simulink model "arducopter"  (R2021a)
settings: Solver=FixedStepAuto  StartTime=0.0  StopTime=simIn.param.timeEnd  FixedStep=simIn.param.dt  RelTol=1e-3
undefined symbols (not defined in the file or in its folder): DiscIntNeverNeededParam, sim, simIn
libraries: simulink x35, slident x4, vrlib x1
(part 7 of 9)

== matlab function arducopter/Attitude Controller/input_euler_angle_roll_pitch_euler_rate_yaw()/Feedforward enabled/input shaping/input shaping roll angle/Square Root Controller1/Square Root Controller ==
  data: err input; correction_rate output; p input; second_ord_lim input; dt input
function correction_rate = sqrt_controller(err, p, second_ord_lim, dt)
% The square root controller
% Code is taken from sqrt_controller(...) in AC_PosControl.cpp.

if (second_ord_lim < 0 || second_ord_lim == 0)
   correction_rate = err * p;
elseif (p == 0)
    % P term is zero, but second order limit is positive
    if (err > 0)
        correction_rate = sqrt(single(2.0) * second_ord_lim * err);
    elseif (err < 0)
        correction_rate = sqrt(single(2.0) * second_ord_lim * -err);
    else
        correction_rate = single(0.0);
    end
else
    % P term and second order limit are positive, hence have been defined
    linear_dist = second_ord_lim / (p * p);
    % Check if error exceeds linear range of controller gain
    if (err > linear_dist)
        correction_rate = sqrt(single(2.0) * second_ord_lim * ( err - (linear_dist / single(2.0)) ));
    elseif (err < -linear_dist)
        correction_rate = -sqrt(single(2.0) * second_ord_lim * ( -err - (linear_dist / single(2.0)) ));
    else
        % Return linearly amplified correction if error is in linear range
        correction_rate = err * p;
    end
end

% Prevent oscillations by over-shooting the error correction in the last
% time step
if (dt ~= 0)
    correction_rate = max( min(correction_rate, abs(err) / dt), -abs(err) / dt);
end

== matlab function arducopter/Attitude Controller/input_euler_angle_roll_pitch_euler_rate_yaw()/Feedforward enabled/input shaping/input shaping yaw rate/Square Root Controller/Square Root Controller ==
  data: err input; correction_rate output; p input; second_ord_lim input; dt input
function correction_rate = sqrt_controller(err, p, second_ord_lim, dt)
% The square root controller
% Code is taken from sqrt_controller(...) in AC_PosControl.cpp.

if (second_ord_lim < 0 || second_ord_lim == 0)
   correction_rate = err * p;
elseif (p == 0)
    % P term is zero, but second order limit is positive
    if (err > 0)
        correction_rate = sqrt(single(2.0) * second_ord_lim * err);
    elseif (err < 0)
        correction_rate = sqrt(single(2.0) * second_ord_lim * -err);
    else
        correction_rate = single(0.0);
    end
else
    % P term and second order limit are positive, hence have been defined
    linear_dist = second_ord_lim / (p * p);
    % Check if error exceeds linear range of controller gain
    if (err > linear_dist)
        correction_rate = sqrt(single(2.0) * second_ord_lim * ( err - (linear_dist / single(2.0)) ));
    elseif (err < -linear_dist)
        correction_rate = -sqrt(single(2.0) * second_ord_lim * ( -err - (linear_dist / single(2.0)) ));
    else
        % Return linearly amplified correction if error is in linear range
        correction_rate = err * p;
    end
end

% Prevent oscillations by over-shooting the error correction in the last
% time step
if (dt ~= 0)
    correction_rate = max( min(correction_rate, abs(err) / dt), -abs(err) / dt);
end

== matlab function arducopter/Throttle/Throttle Calculations/Throttle-Attitude-Mixing/get_throttle_hover/MATLAB Function ==
  data: thrHover input; thrHoverLim output; thrHoverMin input; thrHoverMax input
function thrHoverLim = constrain(thrHover, thrHoverMin, thrHoverMax)

thrHoverLim = min( max( thrHover, thrHoverMin), thrHoverMax);

== matlab function arducopter/Attitude Controller/Determine angleLimit/MATLAB Function2 ==
  data: altholdLeanAngleMax input; altholdLeanAngleMaxCDeg output; angleLimitMin input
function altholdLeanAngleMaxCDeg = get_althold_lean_angle_max_cd(altholdLeanAngleMax, angleLimitMin)
% Based on AC_AttitudeControl::get_althold_lean_angle_max_cd().
% Function calculates a tilt angle limit for pilot input that prioritises
% altitude hold over lean angle.
altholdLeanAngleMaxCDeg = max(180/pi * altholdLeanAngleMax, angleLimitMin) * 100;

== matlab function arducopter/Throttle/Throttle Calculations/MATLAB Function ==
  data: thrThstMax input; throttle_in input; angleLimitTc input; dt input; angleLimitThrMax input; altholdLeanAngleMax_ data_store_memory; altholdLeanAngleMax output
function altholdLeanAngleMax = update_althold_lean_angle_max(thrThstMax, throttle_in, angleLimitTc, dt, angleLimitThrMax)
% Based on AC_AttitudeControl_Multi::update_althold_lean_angle_max. 
% Function updates Althold angle maximum.

global altholdLeanAngleMax_

if thrThstMax == 0
    altholdLeanAngleMax_ = single(0);
    altholdLeanAngleMax = single(0);
    return;
end

altholdLeanAngleMax = acos(min(max(throttle_in / (angleLimitThrMax * thrThstMax), single(0)), single(1)));
altholdLeanAngleMax_ = altholdLeanAngleMax_ + (dt / (dt + angleLimitTc)) * (altholdLeanAngleMax - altholdLeanAngleMax_);
altholdLeanAngleMax = altholdLeanAngleMax_;

== matlab function arducopter/Throttle/Throttle Calculations/Throttle Limiting based on battery state/Update Lift Max from Battery Voltage ==
  data: battVoltFiltLast input; battVoltFilt output single; battVoltRestEst input; liftMax output single; battVoltMax input; battVoltMin input single; thstCurveExpo input; battVoltMinAct output single; battVoltRestEstAct output single; loop_rate input
function [battVoltFilt, liftMax, battVoltMinAct, battVoltRestEstAct] = update_lift_max_from_batt_voltage(battVoltFiltLast, battVoltRestEst, battVoltMax, battVoltMin, thstCurveExpo, loop_rate)
% Code taken from AP_MotorsMulticopter::update_lift_max_from_batt_voltage()
% in AP_MotorsMulticopter.cpp

% Check if batt_volt_min is too small
if (battVoltMax <= 0 || (battVoltMin >= battVoltMax) ...
        || battVoltRestEst < 0.25 * battVoltMin)
    battVoltFilt = single(1.0);
    liftMax = single(1.0);
    battVoltMinAct = battVoltMin;
    battVoltRestEstAct = battVoltRestEst;
    return;
end

% Set lower battery voltage limit for thrust scaling to a new value
battVoltMinAct = max(battVoltMin, battVoltMax * 0.6);

% Constrain resting voltage estimate (resting voltage is actual voltage
% with sag removed based on current draw and resistance)
battVoltRestEstAct = max( min(battVoltRestEst, battVoltMax), battVoltMin);

%% Filter battery voltage at 0.5 Hz. 
% Cutoff Frequency defined in AP_MotorsMulticopter.h
cutoff_freq = single(0.5);
% Calculate time constant and alpha value
T = 1 / (2 * pi * cutoff_freq);
dt = 1 / loop_rate;
alpha = dt / (dt + T);
alpha = max( min( alpha, 1.0), 0.0);

% Filter input is batt_volt_rest_est / batt_volt_comp_max
in = battVoltRestEstAct / battVoltMax;

% Output calculation
battVoltFilt = battVoltFiltLast + (in - battVoltFiltLast) * alpha;

%% Calculate lift_max
thstCurveExpo = max( min(thstCurveExpo, 1), -1);
liftMax = battVoltFilt * (1 - thstCurveExpo) + thstCurveExpo * battVoltFilt * battVoltFilt;

== matlab function arducopter/Throttle/Throttle Calculations/Throttle Limiting based on battery state/Get current throttle limit ==
  data: thrThstMax output; batVoltMin input; batCurrMax input; batCurrT input; loop_rate input; batCurr input; batRes input; batVolt input; thrLimit output; thrHover input; thrLimitLast input single
function [thrThstMax, thrLimit] = get_current_limit_max_throttle(batVoltMin, batCurrMax, batCurrT, loop_rate, batCurr, batRes, batVolt, thrHover, thrLimitLast)
% Code is based on AP_MotorsMulticopter::get_current_limit_max_throttle()
% in AP_MotorsMulticopter.cpp. 
% Returns a throttle limit based on the maximum battery current as a number
% from 0~1 in the range throttle_min to throttle_max.

% Return maximum if current limiting is disabled
if(batCurrMax <= 0) 
    thrLimit = single(1.0);
    thrThstMax = single(1.0);
    return;
end
% Return maximum if battery resistance is not measured
if(batRes == 0)
    thrLimit = single(1.0);
    thrThstMax = single(1.0);
    return;
end

%% Calculate throttle limit
% The throttle limit represents the maximum throttle potential that is left
% based on the actual current compared to the maximum battery current.

% Maximum current to prevent voltage sag below batt_voltage_min
% Since the actual battery current level is used as the minimum for the limit,
% the actual current can still be used to maintain the current throttle. 
batt_curr_max_new = min(batCurrMax, batCurr + (batVolt - batVoltMin) / batRes);
% Calcualte current artion
batt_curr_ratio = batCurr / batt_curr_max_new;
% Calculate time step
dt = 1 / loop_rate;
% Calculate throttle limit as the additional throttle on top of throttle
% hover
thrLimit = thrLimitLast + (dt / (dt + batCurrT)) * (1.0 - batt_curr_ratio);
% Throttle limit drops to 20% between hover an full throttle
thrLimit = max( min( thrLimit, 1.0), 0.2);

% Calculate maximum throttle as sum of hover throttle and the possible
% additional throttle based on the maximum current.
thrThstMax = thrHover + ((1.0 - thrHover) * thrLimit);

== matlab function arducopter/Rate Controller/PID Yaw Rate/I/Integrator ==
  data: error input; integrator_out output; integrator input single; limit_flg input; ki input; i_max input; dt input
function integrator_out = fcn(error, integrator, limit_flg, ki, i_max, dt)
% Code is based on AC_PID::update_i() in AC_PID.cpp.

% Check plausibility of input parameters
if (ki ~= 0 && dt > 0)
    % Only allow integration if limit is not set or the absolute sum of the
    % integrator would be reduced.
    if (~limit_flg || (integrator > 0 && error < 0) || (integrator < 0 && error > 0))
        integrator_out = integrator + error * ki * dt;
        integrator_out = max( min(integrator_out, i_max), -i_max);
    else % Otherwise, keep old integrator value
        integrator_out = integrator;
    end
else % Reset integrator if input parameters are not plausible
    integrator_out = single(0.0);
end

== matlab function arducopter/Rate Controller/PID Roll Rate/I/Integrator ==
  data: error input; integrator_out output; integrator input single; limit_flg input; ki input; i_max input; dt input
function integrator_out = fcn(error, integrator, limit_flg, ki, i_max, dt)
% Code is based on AC_PID::update_i() in AC_PID.cpp.

% Check plausibility of input parameters
if (ki ~= 0 && dt > 0)
    % Only allow integration if limit is not set or the absolute sum of the
    % integrator would be reduced.
    if (~limit_flg || (integrator > 0 && error < 0) || (integrator < 0 && error > 0))
        integrator_out = integrator + error * ki * dt;
        integrator_out = max( min(integrator_out, i_max), -i_max);
    else % Otherwise, keep old integrator value
        integrator_out = integrator;
    end
else % Reset integrator if input parameters are not plausible
    integrator_out = single(0.0);
end

== matlab function arducopter/Throttle/Throttle Calculations/Get compensation gain ==
  data: liftMax input; compGain output single; airDensityRatio input
function compGain = fcn(liftMax, airDensityRatio)
% Code is based on AP_MotorsMulticopter::get_compensation_gain() in
% AP_MotorsMulticopter.cpp.

% Avoid to divide by zero
if(liftMax <= 0.0)
    compGain = single(1.0);
    return;
end

compGain = 1.0 / liftMax;

% Limit air density ratio
airDensityRatioLim = double(max( min( airDensityRatio, 1.25 ), 0.5));

if (airDensityRatio > 0.3 && airDensityRatio < 1.5)
   compGain = compGain * (1.0 / airDensityRatioLim); 
end

== matlab function arducopter/Rate Controller/PID Roll Rate/Slew Limiter/Calculate Dmod ==
  data: slew_rate input; Dmod output single; sr_max input; sr_tau input; dt input; time input; pos_event_idx data_store_memory; pos_event_stored data_store_memory; pos_event_ms data_store_memory; neg_event_idx data_store_memory; neg_event_stored data_store_memory; neg_event_ms data_store_memory; modifier_slew_rate data_store_memory; output_slew_rate data_store_memory; max_neg_slew_event_ms data_store_memory; max_pos_slew_event_ms data_store_memory; max_neg_slew_rate data_store_memory; max_pos_slew_rate data_store_memory
function Dmod   = fcn(slew_rate, sr_max, sr_tau, dt, time)
% Code is based on SlewLimiter::modifier() in SlewLimiter.cpp. 

% Define global variables, so that quanitities do not have to be fed back
% to the function
global pos_event_stored;
global pos_event_idx;
global pos_event_ms;
global max_pos_slew_rate;
global max_pos_slew_event_ms;
global neg_event_stored;
global neg_event_idx;
global neg_event_ms;
global max_neg_slew_rate;
global max_neg_slew_event_ms;
global modifier_slew_rate;
global output_slew_rate;

% Definition of constants as done in SlewLimiter.h
N_EVENTS = uint32(3); % Number of positive and negative consecutive slew rate exceedance events recorded. Set to 3 because of 1-based indexing.
WINDOW_MS = uint32(300); % Time in ms required for half a cycle of the slowest oscillation frequency expected
MODIFIER_GAIN = 1.5; % Ratio of modifier reduction to slew rate exceedance

% Check if slew limiter is activated
if(sr_max <= 0)
   Dmod = single(1.0);
end

now_ms = uint32(time);
decay_alpha = min(dt, sr_tau) / sr_tau;

%% Save exceedance events in event time vector
% Store a series of positive slew rate exceedance events
if (~pos_event_stored && slew_rate > sr_max)
    if (pos_event_idx >= N_EVENTS)
        pos_event_idx(:) = 1;
    end
    pos_event_ms(pos_event_idx) = now_ms;
    pos_event_idx(:) = pos_event_idx + 1;
    pos_event_stored = true;
    neg_event_stored = false;
end

% Store a series of negative slew rate exceedance events
if (~neg_event_stored && slew_rate < -sr_max)
    if (neg_event_idx >= N_EVENTS)
        neg_event_idx(:) = 1;
    end
    neg_event_ms(neg_event_idx) = now_ms;
    neg_event_idx(:) = neg_event_idx + 1;
    pos_event_stored = false;
    neg_event_stored = true;
end

% Find oldest event time
oldest_ms = now_ms;
for i=1:N_EVENTS-1
   if (pos_event_ms(i) < oldest_ms)
       oldest_ms = pos_event_ms(i);
   end
   if (neg_event_ms(i) < oldest_ms)
       oldest_ms = neg_event_ms(i);
   end
end

%% Calculate maximum slew rate
% Save new maximum slew rates, if oldest maximum is exceeded
% OR decay the peak slew rates (pos. and neg.) if they are outside the
% observed time window
if (slew_rate > max_pos_slew_rate)
    max_pos_slew_rate(:) = min(slew_rate, 10 * sr_max);
    max_pos_slew_event_ms = now_ms;
elseif (now_ms - max_pos_slew_event_ms > WINDOW_MS)
    max_pos_slew_rate = max_pos_slew_rate * (1.0 - decay_alpha);
end

if (slew_rate < -max_neg_slew_rate)
    max_neg_slew_rate(:) = min(-slew_rate, 10 * sr_max);
    max_neg_slew_event_ms = now_ms;
elseif (now_ms - max_neg_slew_event_ms > WINDOW_MS)
    max_neg_slew_rate = max_neg_slew_rate * (1.0 - decay_alpha);
end

% Calculate the averaged maximum slew rate
raw_slew_rate = 0.5 * (max_pos_slew_rate + max_neg_slew_rate);

% When the oldest exceedance event falls outside of the window required for
% the number of exceedance events, apply a further reduction to the maximum
% slew rate. This prevents unwanted gain reductions caused by spikes in the
% demanded angular rates due to changed control modes or similar causes.
modifier_input = raw_slew_rate;
if(now_ms - oldest_ms > N_EVENTS * WINDOW_MS) % no incrementation of N_EVENTS because of 1 based indexing
   oldest_time_from_window = single(0.001) * single(now_ms - oldest_ms - N_EVENTS * WINDOW_MS); 
   modifier_input = modifier_input * single(exp(-oldest_time_from_window / sr_tau));
end

%% Calculation of modifier and output slew rate

% Apply filter to slew rate in order to reduce effects of large setpoint
% changes
attack_alpha = min(2.0 * decay_alpha, 1.0);

modifier_slew_rate = modifier_slew_rate + (modifier_input - modifier_slew_rate) * attack_alpha;
modifier_slew_rate = min(modifier_slew_rate, modifier_input);

output_slew_rate = output_slew_rate + (raw_slew_rate - output_slew_rate) * attack_alpha;
output_slew_rate = min(raw_slew_rate, output_slew_rate);

% Calculate modifier. Only has an impact if sr_max is exceeded by averaged
% slew rate.
if(modifier_slew_rate > sr_max)
    Dmod(:) = sr_max / (sr_max + MODIFIER_GAIN * (modifier_slew_rate - sr_max));
else
    Dmod(:) = 1.0;
end

== matlab function arducopter/Rate Controller/PID Roll Rate/Slew Limiter/Lowpass Filter ==
  data: in input; out output single; cutoff_freq input; loop_rate input; out_last input
function out  = fcn(in, cutoff_freq, loop_rate, out_last)
% The code is based on the apply(sample, cutoff_freq, dt) function in
% LowPassFilter.cpp
dt = 1 / loop_rate;

% Check if filter is supposed to be filtering
if (cutoff_freq <=0 || dt <= 0)
    out = in;
    return;
end

% Calculate time constant and alpha value
T = 1 / (2 * pi * cutoff_freq);
alpha = dt / (dt + T);
alpha = max( min( alpha, 1.0), 0.0);

% Output calculation
out = out_last + (in - out_last) * alpha;

== matlab function arducopter/Throttle/Throttle Calculations/Air density Calculation/Get equivalent to true airspeed EAS2TAS ==
  data: alt input; eas2tas output; airPress input; gndTemp input; EAS2TAS data_store_memory; last_alt_EAS2TAS data_store_memory
function eas2tas = fcn(alt, airPress, gndTemp)
% Code is based on AP_Baro::get_EAS2TAS() in AP_Baro.cpp.

% Constants
C_TO_KELVIN = single(273.15); % Conversion offset from celsius to kelvin
ISA_LAPSE_RATE = single(0.0065);
ISA_GAS_CONSTANT = single(287.26);
SSL_AIR_DENSITY = single(1.225);

% Global variables
global EAS2TAS;
global last_alt_EAS2TAS;

% Check if altitude has changed significally
if ((abs(alt - last_alt_EAS2TAS) < 25.0) && EAS2TAS ~= 0)
    % Change too small to require re-calculating
   eas2tas = EAS2TAS;
   return;
end

if (airPress == 0)
   eas2tas = single(1.0);
   return;
end

tempK = single(gndTemp + C_TO_KELVIN - ISA_LAPSE_RATE * alt);
eas2tas_squared = SSL_AIR_DENSITY / (airPress / (ISA_GAS_CONSTANT * tempK));
if (eas2tas_squared <= 0)
    eas2tas = single(1.0);
    return;
end
EAS2TAS = sqrt(eas2tas_squared);
last_alt_EAS2TAS = alt;
eas2tas = EAS2TAS;

== matlab function arducopter/Throttle/Throttle Calculations/Air density Calculation/Get air density ratio ==
  data: eas2tas input; airDensityRatio output
function airDensityRatio = fcn(eas2tas)
% Code is based on AP_Baro::get_air_density_ratio() in AP_Baro.cpp.
if (eas2tas > 0.0)
    airDensityRatio = single(1.0 / (eas2tas*eas2tas));
else
    airDensityRatio = single(1.0);
end

== matlab function arducopter/Attitude Controller/input_euler_angle_roll_pitch_euler_rate_yaw()/Feedforward enabled/input shaping/input shaping pitch angle/MATLAB Function1 ==
  data: desiredAngVel input; targetAngVel input; eulerRateTar output; accelMax input; dt input; input_tc input
function eulerRateTar = input_shaping_ang_vel(desiredAngVel, targetAngVel, accelMax, dt, input_tc)
% Limits acceleration and deceleration of a velocity request
% Code based on AC_AttitudeControl::input_shaping_ang_vel()

if input_tc > 0
    % Calculate the acceleration to smoothly achieve rate. Jerk is not limited.
    errorRate = desiredAngVel - targetAngVel;
    desiredAngAccel = sqrt_controller(errorRate, 1.0/max(input_tc, single(0.01)), single(0), dt);
    desiredAngVel = targetAngVel + desiredAngAccel * dt;
end

% Acceleration is limited directly to smooth the beginning of the curve
if accelMax > 0
    deltaAngVel = accelMax * dt;
    eulerRateTar = min(max(desiredAngVel, targetAngVel - deltaAngVel), targetAngVel + deltaAngVel);
else
    eulerRateTar = desiredAngVel;
end

== matlab function arducopter/Attitude Controller/input_euler_angle_roll_pitch_euler_rate_yaw()/Feedforward enabled/input shaping/input shaping yaw rate/MATLAB Function1 ==
  data: desiredAngVel input; targetAngVel input; eulerRateTar output; accelMax input; dt input; input_tc input
function eulerRateTar = input_shaping_ang_vel(desiredAngVel, targetAngVel, accelMax, dt, input_tc)
% Limits acceleration and deceleration of a velocity request
% Code based on AC_AttitudeControl::input_shaping_ang_vel()

if input_tc > 0
    % Calculate the acceleration to smoothly achieve rate. Jerk is not limited.
    errorRate = desiredAngVel - targetAngVel;
    desiredAngAccel = sqrt_controller(errorRate, 1.0/max(input_tc, single(0.01)), single(0), dt);
    desiredAngVel = targetAngVel + desiredAngAccel * dt;
end

% Acceleration is limited directly to smooth the beginning of the curve
if accelMax > 0
    deltaAngVel = accelMax * dt;
    eulerRateTar = min(max(desiredAngVel, targetAngVel - deltaAngVel), targetAngVel + deltaAngVel);
else
    eulerRateTar = desiredAngVel;
end

== matlab function arducopter/Rate Controller/PID Yaw Rate/Slew Limiter/Calculate Dmod ==
  data: slew_rate input; Dmod output single; sr_max input; sr_tau input; dt input; time input; pos_event_idx data_store_memory; pos_event_stored data_store_memory; pos_event_ms data_store_memory; neg_event_idx data_store_memory; neg_event_stored data_store_memory; neg_event_ms data_store_memory; modifier_slew_rate data_store_memory; output_slew_rate data_store_memory; max_neg_slew_event_ms data_store_memory; max_pos_slew_event_ms data_store_memory; max_neg_slew_rate data_store_memory; max_pos_slew_rate data_store_memory
function Dmod   = fcn(slew_rate, sr_max, sr_tau, dt, time)
% Code is based on SlewLimiter::modifier() in SlewLimiter.cpp. 

% Define global variables, so that quanitities do not have to be fed back
% to the function
global pos_event_stored;
global pos_event_idx;
global pos_event_ms;
global max_pos_slew_rate;
global max_pos_slew_event_ms;
global neg_event_stored;
global neg_event_idx;
global neg_event_ms;
global max_neg_slew_rate;
global max_neg_slew_event_ms;
global modifier_slew_rate;
global output_slew_rate;

% Definition of constants as done in SlewLimiter.h
N_EVENTS = uint32(3); % Number of positive and negative consecutive slew rate exceedance events recorded. Set to 3 because of 1-based indexing.
WINDOW_MS = uint32(300); % Time in ms required for half a cycle of the slowest oscillation frequency expected
MODIFIER_GAIN = 1.5; % Ratio of modifier reduction to slew rate exceedance

% Check if slew limiter is activated
if(sr_max <= 0)
   Dmod = single(1.0);
end

now_ms = uint32(time);
decay_alpha = min(dt, sr_tau) / sr_tau;

%% Save exceedance events in event time vector
% Store a series of positive slew rate exceedance events
if (~pos_event_stored && slew_rate > sr_max)
    if (pos_event_idx >= N_EVENTS)
        pos_event_idx(:) = 1;
    end
    pos_event_ms(pos_event_idx) = now_ms;
    pos_event_idx(:) = pos_event_idx + 1;
    pos_event_stored = true;
    neg_event_stored = false;
end

% Store a series of negative slew rate exceedance events
if (~neg_event_stored && slew_rate < -sr_max)
    if (neg_event_idx >= N_EVENTS)
        neg_event_idx(:) = 1;
    end
    neg_event_ms(neg_event_idx) = now_ms;
    neg_event_idx(:) = neg_event_idx + 1;
    pos_event_stored = false;
    neg_event_stored = true;
end

% Find oldest event time
oldest_ms = now_ms;
for i=1:N_EVENTS-1
   if (pos_event_ms(i) < oldest_ms)
       oldest_ms = pos_event_ms(i);
   end
   if (neg_event_ms(i) < oldest_ms)
       oldest_ms = neg_event_ms(i);
   end
end

%% Calculate maximum slew rate
% Save new maximum slew rates, if oldest maximum is exceeded
% OR decay the peak slew rates (pos. and neg.) if they are outside the
% observed time window
if (slew_rate > max_pos_slew_rate)
    max_pos_slew_rate(:) = min(slew_rate, 10 * sr_max);
    max_pos_slew_event_ms = now_ms;
elseif (now_ms - max_pos_slew_event_ms > WINDOW_MS)
    max_pos_slew_rate = max_pos_slew_rate * (1.0 - decay_alpha);
end

if (slew_rate < -max_neg_slew_rate)
    max_neg_slew_rate(:) = min(-slew_rate, 10 * sr_max);
    max_neg_slew_event_ms = now_ms;
elseif (now_ms - max_neg_slew_event_ms > WINDOW_MS)
    max_neg_slew_rate = max_neg_slew_rate * (1.0 - decay_alpha);
end

% Calculate the averaged maximum slew rate
raw_slew_rate = 0.5 * (max_pos_slew_rate + max_neg_slew_rate);

% When the oldest exceedance event falls outside of the window required for
% the number of exceedance events, apply a further reduction to the maximum
% slew rate. This prevents unwanted gain reductions caused by spikes in the
% demanded angular rates due to changed control modes or similar causes.
modifier_input = raw_slew_rate;
if(now_ms - oldest_ms > N_EVENTS * WINDOW_MS) % no incrementation of N_EVENTS because of 1 based indexing
   oldest_time_from_window = single(0.001) * single(now_ms - oldest_ms - N_EVENTS * WINDOW_MS); 
   modifier_input = modifier_input * single(exp(-oldest_time_from_window / sr_tau));
end

%% Calculation of modifier and output slew rate

% Apply filter to slew rate in order to reduce effects of large setpoint
% changes
attack_alpha = min(2.0 * decay_alpha, 1.0);

modifier_slew_rate = modifier_slew_rate + (modifier_input - modifier_slew_rate) * attack_alpha;
modifier_slew_rate = min(modifier_slew_rate, modifier_input);

output_slew_rate = output_slew_rate + (raw_slew_rate - output_slew_rate) * attack_alpha;
output_slew_rate = min(raw_slew_rate, output_slew_rate);

% Calculate modifier. Only has an impact if sr_max is exceeded by averaged
% slew rate.
if(modifier_slew_rate > sr_max)
    Dmod(:) = sr_max / (sr_max + MODIFIER_GAIN * (modifier_slew_rate - sr_max));
else
    Dmod(:) = 1.0;
end

== matlab function arducopter/Rate Controller/PID Yaw Rate/Slew Limiter/Lowpass Filter ==
  data: in input; out output single; cutoff_freq input; loop_rate input; out_last input
function out  = fcn(in, cutoff_freq, loop_rate, out_last)
% The code is based on the apply(sample, cutoff_freq, dt) function in
% LowPassFilter.cpp
dt = 1 / loop_rate;

% Check if filter is supposed to be filtering
if (cutoff_freq <=0 || dt <= 0)
    out = in;
    return;
end

% Calculate time constant and alpha value
T = 1 / (2 * pi * cutoff_freq);
alpha = dt / (dt + T);
alpha = max( min( alpha, 1.0), 0.0);

% Output calculation
out = out_last + (in - out_last) * alpha;

== matlab function arducopter/Position Controller/PID Velocity z/I/Integrator ==
  data: error input; integrator_out output; integrator input single; limitNeg input; limitPos input; ki input; i_max input; dt input
function integrator_out = fcn(error, integrator, limitNeg, limitPos, ki, i_max, dt)
% Code is based on AC_PID_Basic::update_i() in AC_PID_Basic.

% Check plausibility of input parameters
if (ki ~= 0)
    % Integration can only be executed if limits are not exceeded or if
    % limits are exceeded but the current error would reduce output
    if (~((limitNeg && error < 0) || (limitPos && error > 0)))
        integrator_out = integrator + error * ki * dt;
        integrator_out = max( min(integrator_out, i_max), -i_max);
    else % Otherwise, keep old integrator value
        integrator_out = integrator;
    end
else % Reset integrator if input parameters are not plausible
    integrator_out = single(0.0);
end

== matlab function arducopter/Position Controller/PID Acceleration z/I/Integrator ==
  data: error input; integrator_out output; integrator input single; limit_flg input; ki input; i_max input; dt input
function integrator_out = fcn(error, integrator, limit_flg, ki, i_max, dt)
% Code is based on AC_PID::update_i() in AC_PID, line 230.

% Check plausibility of input parameters
if (ki ~= 0 && dt > 0)
    % Only allow integration if limit is not set or the absolute sum of the
    % integrator would be reduced.
    if (~limit_flg || (integrator > 0 && error < 0) || (integrator < 0 && error > 0))
        integrator_out = integrator + error * ki * dt;
        integrator_out = max( min(integrator_out, i_max), -i_max);
    else % Otherwise, keep old integrator value
        integrator_out = integrator;
    end
else % Reset integrator if input parameters are not plausible
    integrator_out = single(0.0);
end

== matlab function arducopter/Position Controller/PID Acceleration z/Slew Limiter/Calculate Dmod ==
  data: slew_rate input; Dmod output single; sr_max input; sr_tau input; dt input; time input; pos_event_idx data_store_memory; pos_event_stored data_store_memory; pos_event_ms data_store_memory; neg_event_idx data_store_memory; neg_event_stored data_store_memory; neg_event_ms data_store_memory; modifier_slew_rate data_store_memory; output_slew_rate data_store_memory; max_neg_slew_event_ms data_store_memory; max_pos_slew_event_ms data_store_memory; max_neg_slew_rate data_store_memory; max_pos_slew_rate data_store_memory
function Dmod   = fcn(slew_rate, sr_max, sr_tau, dt, time)
% Code is based on SlewLimiter::modifier() in SlewLimiter.cpp. 

% Define global variables, so that quanitities do not have to be fed back
% to the function
global pos_event_stored;
global pos_event_idx;
global pos_event_ms;
global max_pos_slew_rate;
global max_pos_slew_event_ms;
global neg_event_stored;
global neg_event_idx;
global neg_event_ms;
global max_neg_slew_rate;
global max_neg_slew_event_ms;
global modifier_slew_rate;
global output_slew_rate;

% Definition of constants as done in SlewLimiter.h
N_EVENTS = uint32(3); % Number of positive and negative consecutive slew rate exceedance events recorded. Set to 3 because of 1-based indexing.
WINDOW_MS = uint32(300); % Time in ms required for half a cycle of the slowest oscillation frequency expected
MODIFIER_GAIN = 1.5; % Ratio of modifier reduction to slew rate exceedance

% Check if slew limiter is activated
if(sr_max <= 0)
   Dmod = single(1.0);
end

now_ms = uint32(time);
decay_alpha = min(dt, sr_tau) / sr_tau;

%% Save exceedance events in event time vector
% Store a series of positive slew rate exceedance events
if (~pos_event_stored && slew_rate > sr_max)
    if (pos_event_idx >= N_EVENTS)
        pos_event_idx(:) = 1;
    end
    pos_event_ms(pos_event_idx) = now_ms;
    pos_event_idx(:) = pos_event_idx + 1;
    pos_event_stored = true;
    neg_event_stored = false;
end

% Store a series of negative slew rate exceedance events
if (~neg_event_stored && slew_rate < -sr_max)
    if (neg_event_idx >= N_EVENTS)
        neg_event_idx(:) = 1;
    end
    neg_event_ms(neg_event_idx) = now_ms;
    neg_event_idx(:) = neg_event_idx + 1;
    pos_event_stored = false;
    neg_event_stored = true;
end

% Find oldest event time
oldest_ms = now_ms;
for i=1:N_EVENTS-1
   if (pos_event_ms(i) < oldest_ms)
       oldest_ms = pos_event_ms(i);
   end
   if (neg_event_ms(i) < oldest_ms)
       oldest_ms = neg_event_ms(i);
   end
end

%% Calculate maximum slew rate
% Save new maximum slew rates, if oldest maximum is exceeded
% OR decay the peak slew rates (pos. and neg.) if they are outside the
% observed time window
if (slew_rate > max_pos_slew_rate)
    max_pos_slew_rate(:) = min(slew_rate, 10 * sr_max);
    max_pos_slew_event_ms = now_ms;
elseif (now_ms - max_pos_slew_event_ms > WINDOW_MS)
    max_pos_slew_rate = max_pos_slew_rate * (1.0 - decay_alpha);
end

if (slew_rate < -max_neg_slew_rate)
    max_neg_slew_rate(:) = min(-slew_rate, 10 * sr_max);
    max_neg_slew_event_ms = now_ms;
elseif (now_ms - max_neg_slew_event_ms > WINDOW_MS)
    max_neg_slew_rate = max_neg_slew_rate * (1.0 - decay_alpha);
end

% Calculate the averaged maximum slew rate
raw_slew_rate = 0.5 * (max_pos_slew_rate + max_neg_slew_rate);

% When the oldest exceedance event falls outside of the window required for
% the number of exceedance events, apply a further reduction to the maximum
% slew rate. This prevents unwanted gain reductions caused by spikes in the
% demanded angular rates due to changed control modes or similar causes.
modifier_input = raw_slew_rate;
if(now_ms - oldest_ms > N_EVENTS * WINDOW_MS) % no incrementation of N_EVENTS because of 1 based indexing
   oldest_time_from_window = single(0.001) * single(now_ms - oldest_ms - N_EVENTS * WINDOW_MS); 
   modifier_input = modifier_input * single(exp(-oldest_time_from_window / sr_tau));
end

%% Calculation of modifier and output slew rate

% Apply filter to slew rate in order to reduce effects of large setpoint
% changes
attack_alpha = min(2.0 * decay_alpha, 1.0);

modifier_slew_rate = modifier_slew_rate + (modifier_input - modifier_slew_rate) * attack_alpha;
modifier_slew_rate = min(modifier_slew_rate, modifier_input);

output_slew_rate = output_slew_rate + (raw_slew_rate - output_slew_rate) * attack_alpha;
output_slew_rate = min(raw_slew_rate, output_slew_rate);

% Calculate modifier. Only has an impact if sr_max is exceeded by averaged
% slew rate.
if(modifier_slew_rate > sr_max)
    Dmod(:) = sr_max / (sr_max + MODIFIER_GAIN * (modifier_slew_rate - sr_max));
else
    Dmod(:) = 1.0;
end

== matlab function arducopter/Motor Mixer/Calculate motor thrust ==
  data: roll input; limitRoll output; limitPitch output; pitch input; yaw input; thrIn input; thrAvgMax input; thrThstMaxIn input; compGain input; yawHeadroom input; numMotors input; facMotors input; limitYaw output; limitThrLower output; limitThrUpper output; thrOut output; thstOut output; thst_rpyt data_store_memory
function [limitRoll, limitPitch, limitYaw, limitThrLower, limitThrUpper, thrOut, thstOut] = outputArmedStabilizing(roll, pitch, yaw, thrIn, thrAvgMax, thrThstMaxIn, compGain, yawHeadroom, numMotors, facMotors)
% The calculation is taken from output_armed_stabilizing() in
% AP_MotorsMatrix.cpp.
% Contrary to the original code, lost motors are not considered

global thst_rpyt;

%% Preperations
% Definitions
roll_factor = facMotors(1,:);              % Factors of motors for thrust on differen axis - needs to moved to Init-file, together with calculation
pitch_factor = facMotors(2,:);
yaw_factor = facMotors(3,:);
throttle_factor = facMotors(4,:);
limitRoll = false;                             % Initialize limit flags to prevent missing assignment error of Simulink
limitPitch = false;
limitYaw = false;
limitThrLower = false;
limitThrUpper = false;
yaw_allowed = single(1.0);                          % Amount of yaw that can be realized
rpy_scale = single(1.0);                            % Scale factor to fit roll, pitch and yaw within motor limits
throttle_thrust_best_rpy = single(0.0);             % Amount of throttle that provides maximum roll, pitch and yaw without climbing                      
thrust_boost_ratio = single(0.0);                   % Ratio for thrust boosting in case of a motor failure. Set to 0 for normal operation!     

% TODO: Voltage and air pressure compensation
roll_thrust = roll * compGain;
pitch_thrust = pitch * compGain;
yaw_thrust = yaw * compGain;
throttle_thrust = thrIn * compGain;             % Pilot's desired throttle
thrAvgMax = thrAvgMax * compGain;

% Calculate maximum throttle thrust input value
throttle_thrust_max = thrust_boost_ratio + (1.0 - thrust_boost_ratio) * thrThstMaxIn;

% Sanity check: Throttle above zero and below current limnited throttle.
% Limit Throttle otherwise
if (throttle_thrust <= 0)
    throttle_thrust = single(0.0);
    limitThrLower = true;
end
if (throttle_thrust >= throttle_thrust_max)
    throttle_thrust = throttle_thrust_max;
    limitThrUpper = true;
end
% Limit throttle average max
thrAvgMax = max( min( thrAvgMax, throttle_thrust_max), throttle_thrust);
% Calculate highest allowed average throttle that will provide maximum
% control range of roll, pitch and yaw without climbing
throttle_thrust_best_rpy = min(single(0.5), thrAvgMax);

%% Calculation of the throttle that gives most room for yaw
% This corresponds to the lower of
%   1. 0.5 - (rpy_low + rpy_high) / 2.0) --> This gives the maximum
%   possible margin above the highest motor and below the lowest
%   2. The higher of
%       a) Pilots throttle input
%       b) The point throttle_rpy_mix between pilot's input throttle and
%       hover throttle

% First: Calculate amount of yaw that fits into throttle range
rp_low = single(1.0);
rp_high = single(-1.0);
for i=1:numMotors
    % Combined thrust output of roll and pitch
    thst_rpyt(i) = roll_thrust * roll_factor(i) + pitch_thrust * pitch_factor(i); 
    
    % Record lowest thrust command
    if (thst_rpyt(i) < rp_low)
        rp_low = thst_rpyt(i);
    end
    % Record highest thrust command
    if (thst_rpyt(i) > rp_high)
        rp_high = thst_rpyt(i);
    end
    
    % Check maximum yaw control that can be used
    if(yaw_factor(i)~=0)
        if ((yaw_thrust * yaw_factor(i)) > 0)
           yaw_allowed = min(yaw_allowed, abs( max(1.0 - throttle_thrust_best_rpy + thst_rpyt(i), 0.0)/yaw_factor(i) ) ); 
        else
           yaw_allowed = min(yaw_allowed, abs( max(throttle_thrust_best_rpy + thst_rpyt(i), 0.0)/yaw_factor(i) ) );
        end
    end    
end

% Calculate the maximum yaw control that can be used
yaw_allowed_min = yawHeadroom / 1000.0;
% If thrust boost is enabled, increase headroom to 50%
yaw_allowed_min = thrust_boost_ratio * 0.5 + (1.0 - thrust_boost_ratio) * yaw_allowed_min;

yaw_allowed = max(yaw_allowed, yaw_allowed_min);

%% Add yaw control to thrust outputs
% Limit yaw thrust to allowed range
if (abs(yaw_thrust) > yaw_allowed)
    yaw_thrust = min( max(-yaw_allowed, yaw_thrust), yaw_allowed);
    limitYaw = true;
end

rpy_low = single(1.0);
rpy_high = single(-1.0);
for i=1:numMotors
    % Combined thrust command for roll, pitch and yaw
   thst_rpyt(i) = thst_rpyt(i) + yaw_thrust * yaw_factor(i);
   
   % Record lowest thrust command
    if (thst_rpyt(i) < rpy_low)
        rpy_low = thst_rpyt(i);
    end
    % Record highest thrust command
    if (thst_rpyt(i) > rpy_high)
        rpy_high = thst_rpyt(i);
    end
end

%% Scale outputs
% Calculate any sclaing that is needed to fit combined thrust outputs
% within the output range
if (rpy_high - rpy_low > 1.0)
    rpy_scale(:) = 1.0 / (rpy_high-rpy_low);
end
if (thrAvgMax + rpy_low < 0)
    rpy_scale(:) = min(rpy_scale, -thrAvgMax / rpy_low);
end

% Calculate how close the motors can come to the desired throttle
rpy_high = rpy_high * rpy_scale;
rpy_low = rpy_low * rpy_scale;
throttle_thrust_best_rpy = -rpy_low;
% Calculate the difference between pilot's desired throttle and
% throttle_thrust_best_rpy
thr_adj = single(throttle_thrust - throttle_thrust_best_rpy);
if (rpy_scale < 1.0) % Full range of throttle is already being used
    limitRoll(:) = true;
    limitPitch(:) = true;
    limitYaw(:) = true;
    if (thr_adj > 0.0)
       limitThrUpper = true; 
    end
    thr_adj(:) = 0.0;
else
    if (thr_adj < 0.0) % Throttle can't be reduced to reach desired value
        thr_adj(:) = 0.0;
    elseif (thr_adj > 1.0 - (throttle_thrust_best_rpy + rpy_high))
       % Throttle can't be increased to desired value
       thr_adj(:) = 1.0 - (throttle_thrust_best_rpy + rpy_high);
       limitThrUpper = true;
    end
end

%% Calculate resulting thrust outputs
% Calculate adjusted throttle value
throttle_thrust_best_plus_adj = throttle_thrust_best_rpy + thr_adj;
% Add scaled roll, pitch, constrained yaw and throttle for each motor
for i=1:numMotors
    % Combined thrust is the sum of the maximum possible desired throttle
    % "throttle_thrust_best_plus_adj" and the needed thrust to realize the
    % desired angular motion "thrust_rpyt_out(i)"
    thst_rpyt(i) = (throttle_thrust_best_plus_adj * throttle_factor(i)) + (rpy_scale * thst_rpyt(i)); 
end

% Calculate throttle thrust after mixing for harmonic notch
thrOut = throttle_thrust_best_plus_adj / compGain;

% Assign thrust output
thstOut = thst_rpyt;

== matlab function arducopter/Position Controller/P Position z/Calculate error ==
  settings: updateMethod=DISCRETE
  data: tar input; tar_new output; err output; act input; err_min input; err_max input
function [tar_new, err] = calc_err(tar, act, err_min, err_max)
% Code based on AC_P_1D::update_all() in AC_P_1D.cpp.
tar_new = tar; % added line to prevent Simulink error for unassigned tar_new
err = tar - act;

% Limit error and recalculate target
if ((err_min < 0) && (err < err_min))
    err = err_min;
    tar_new = act + err;
elseif ((err_max > 0) && (err > err_max))
    err = err_max;
    tar_new = act + err;
end

== matlab function arducopter/Position Controller/P Position z/Set vertical speed & acceleration limit/Set error limits ==
  data: outMin input; errMin output; outMax input; DoutMax input; errMax output; D1max output; D2OutMax input; kp input
function [errMin, errMax, D1max] = setLimits(outMin, outMax, DoutMax, D2OutMax, kp)
% Code taken from AC_P_1D::set_limits() in AC_P_1D.cpp.
% Input parameter D2_out_max is neglected since it is set to zero in
% AC_PosControl::set_correction_speed_accel_z()

errMin = single(0.0);
errMax = single(0.0);
D1max = single(0.0);

if (DoutMax > 0)
   D1max = DoutMax; 
end

% Missing line left out because of parameter D2_out_max being set to 0

% Call the simulink function inv_sqrt_controller(...) from control.cpp,
% line 343 if the conditions apply
if (outMin < 0 && kp > 0)
    errMin = inv_sqrt_controller(outMin, kp, DoutMax);
end

if (outMax > 0 && kp > 0)
    errMax = inv_sqrt_controller(outMax, kp, DoutMax);
end

== matlab function arducopter/Position Controller/P Position z/Set vertical speed & acceleration limit/Inverse Square Root Controller/Inverse Sqrt Controller ==
  data: output input; errLim output; p input; Dmax input
function errLim = inv_sqrt_controller(output, p, Dmax)
% Code taken from inv_sqrt_controller(...) in control.cpp.
% Function calculates the input (error) to the sqrt_controller required to
% achieve a given output

if (Dmax > 0 && p == 0)
    errLim = output * output / (single(2.0) * Dmax);
    return;
end
if ((Dmax < 0 || Dmax == 0) && p ~= 0)
    errLim = output / p;
    return;
end
if ((Dmax < 0 || Dmax == 0) && p == 0)
   errLim = single(0.0);
   return
end

% Calculate the cross-point velocity, at which we switch from calculating the
% controller output using a linear function to a sqrt function
linear_velocity = Dmax / p;
% Use linear function to calculate limit if current velocity is below
% cross-point velocity
if (abs(output) < linear_velocity)
   errLim = output / p;
   return;
end

% Calculate the cross-point distance at which we switch to sqrt function
linear_dist = Dmax / (p*p);
% Calculate the maximum distance error resulting from the velocity and
% acceleration limit
stopping_dist = (linear_dist * single(0.5)) + (output*output) / (single(2.0) * Dmax);
% If output parameter is negative or zero, return negative maximum distance
% error
if (output > 0)
    errLim = stopping_dist;
else
    errLim = -stopping_dist;
end

== matlab function arducopter/Position Controller/P Position z/Square Root Controller ==
  data: err input; correction_rate output; p input; second_ord_lim input; dt input
function correction_rate = sqrt_controller(err, p, second_ord_lim, dt)
% The square root controller
% Code is taken from sqrt_controller(...) in AC_PosControl.cpp.

if (second_ord_lim < 0 || second_ord_lim == 0)
   correction_rate = err * p;
elseif (p == 0)
    % P term is zero, but second order limit is positive
    if (err > 0)
        correction_rate = sqrt(single(2.0) * second_ord_lim * err);
    elseif (err < 0)
        correction_rate = sqrt(single(2.0) * second_ord_lim * -err);
    else
        correction_rate = single(0.0);
    end
else
    % P term and second order limit are positive, hence have been defined
    linear_dist = second_ord_lim / (p * p);
    % Check if error exceeds linear range of controller gain
    if (err > linear_dist)
        correction_rate = sqrt(single(2.0) * second_ord_lim * ( err - (linear_dist / single(2.0)) ));
    elseif (err < -linear_dist)
        correction_rate = -sqrt(single(2.0) * second_ord_lim * ( -err - (linear_dist / single(2.0)) ));
    else
        % Return linearly amplified correction if error is in linear range
        correction_rate = err * p;
    end
end

% Prevent oscillations by over-shooting the error correction in the last
% time step
if (dt ~= 0)
    correction_rate = max( min(correction_rate, abs(err) / dt), -abs(err) / dt);
end

== matlab function arducopter/Position Controller/PID Acceleration z/Slew Limiter/Lowpass Filter ==
  data: in input; out output single; cutoff_freq input; loop_rate input; out_last input
function out  = fcn(in, cutoff_freq, loop_rate, out_last)
% The code is based on the apply(sample, cutoff_freq, dt) function in
% LowPassFilter.cpp
dt = 1 / loop_rate;

% Check if filter is supposed to be filtering
if (cutoff_freq <=0 || dt <= 0)
    out = in;
    return;
end

% Calculate time constant and alpha value
T = 1 / (2 * pi * cutoff_freq);
alpha = dt / (dt + T);
alpha = max( min( alpha, 1.0), 0.0);

% Output calculation
out = out_last + (in - out_last) * alpha;

== matlab function arducopter/Throttle/Throttle Calculations/Throttle-Attitude-Mixing/Update Throttle Mix Des ==
  data: thrTar input; zVelCtrlRatio input; zVelDes input; thrMan input; thrMixDes output; thrMixMin input; thrMixMax input; thrMixMan input
function thrMixDes = updateThrottleMix(thrTar, zVelCtrlRatio, zVelDes, thrMan, thrMixMin, thrMixMax, thrMixMan)
% Sets desired throttle vs attitude priorization based on vehicle state.
% Low values favour pilot/autpilot throttle over attitude control, high
% values favour attitude control over throttle
% Has not effec twhen throttle > hover throttle
% Code: land_detector.cpp, Copter::update_throttle_mix()

if thrMan
    % Manual throttle
    if thrTar <= 0
        % Call to set_throttle_mix_min() set mix to minimum
        thrMixDes = thrMixMin;
    else
        % Call to set_throttle_mix_man() sets mix to value for manual
        % throttle
        thrMixDes = thrMixMan;
    end
else
    % Autopilot controlled throttle
    
    % Check for aggressive flight request - Requested roll/pitch angle
    % above 15 degrees
    % ToDo

    % Check for large external disturbances - angle error over 30 degrees
    % ToDo

    % Check for large acceleration - falling for high turbulence
    % ToDo

    % Check for requested descent
    descent_not_demanded = zVelDes >= single(0.0);

    if (descent_not_demanded)
        % Call to AC_AttitudeControl_Multi::set_throttle_mix_max(ratio)
        ratio = min( max(single(0.0), zVelCtrlRatio), single(1.0) );
        thrMixDes = (single(1.0) - ratio) * thrMixMin + ratio * thrMixMax;
    else
        thrMixDes = thrMixMin;
    end
end

== matlab function arducopter/Position Controller/zVelCtrlRatio Calculation/Update vel_z_ctrl_ratio ==
  data: velErr input; zVelCtrlRat output; dnVelMax input; dt input; vel_z_ctrl_ratio data_store_memory
function zVelCtrlRat = setZVelCtrlRatio(velErr, dnVelMax, dt)
% Sets vel_z_control_ratio, which contains the proportion of the z velocity
% error relative to the maximum request. Needed in function
% Copter::update_throttle_mix().
% Code: AC_PosControl.cpp, update_z_controller()

global vel_z_ctrl_ratio;

err_ratio = velErr / dnVelMax;
vel_z_ctrl_ratio = vel_z_ctrl_ratio + dt * single(0.1) * (0.5 - err_ratio);
vel_z_ctrl_ratio = min( max(single(0.0), vel_z_ctrl_ratio), single(2.0) );

zVelCtrlRat = vel_z_ctrl_ratio;

== matlab function arducopter/Position Controller/Vertical Speed and Acceleration Limits ==
  data: dnSpeedMax input; upSpeedMax input; zAccMax input; vel_max_down_cms data_store_memory; vel_max_up_cms data_store_memory; acc_max_z_cmss data_store_memory; jerk_max_z_cmsss data_store_memory; zJerkMax input; GRAVITY_MSS input; zAccFltt_f input; zAccFlte_f input
function setMaxSpeedAccelZ(dnSpeedMax, upSpeedMax, zAccMax, zJerkMax, GRAVITY_MSS, zAccFltt_f, zAccFlte_f)
% Sets the maximum vertical speed in cm/s and acceleration in cm/s/s.
% Checks max vertical jerk limits.
% Code: AC_PosControl.cpp, set_max_speed_accel_z().

global vel_max_down_cms;
global vel_max_up_cms;
global acc_max_z_cmss;
global jerk_max_z_cmsss;

% Make sure maximum descending speed is negative
dnSpeedMax = dnSpeedMax * single(-1);

% Sanity check
if dnSpeedMax < 0
    vel_max_down_cms = dnSpeedMax;
end
if upSpeedMax > 0
    vel_max_up_cms = upSpeedMax;
end
if zAccMax > 0
    acc_max_z_cmss = zAccMax;
end

% Ensure that vertical jerk is not limited by filter of z acceleration PID
jerk_max_z_cmsss = single(100) * zJerkMax;
if (zAccFltt_f > 0)
    jerk_max_z_cmsss = min( jerk_max_z_cmsss, min(GRAVITY_MSS * single(100), acc_max_z_cmss) * (2*pi*zAccFltt_f) / single(5.0) );
end
if (zAccFlte_f > 0)
    jerk_max_z_cmsss = min( jerk_max_z_cmsss, min(GRAVITY_MSS * single(100), acc_max_z_cmss) * (2*pi*zAccFlte_f) / single(5.0) );
end

== matlab function arducopter/Lowpass2p/Lowpass Pitch/Lowpass2p ==
  data: u input; y output; sampleFreq input; cutoffFreq input; delElem1 data_store_memory; delElem2 data_store_memory
function y = lowpass2p(u, sampleFreq, cutoffFreq)
% Lowpass filter of order two
% Source: LowPassFilter2p.cpp
global delElem1
global delElem2

% Calculate parameters: LowPassFilter2p.cpp, compute_params()
fr = single(sampleFreq/cutoffFreq);
ohm = single(tan(pi/fr));
c = single(1+2*cos(pi/4)*ohm + ohm*ohm);

b0 = ohm*ohm/c;
b1 = 2*b0;
b2 = b0;
a1 = 2*(ohm*ohm-1)/c;
a2 = single((1-2*cos(pi/4)*ohm+ohm*ohm)/c);

% Calculation of filtered sample: LowPassFilter2p.cpp, apply()
delElem0 = u - delElem1 * a1 - delElem2 * a2;
y = delElem0 * b0 + delElem1 * b1 + delElem2 * b2;

delElem2 = delElem1;
delElem1 = delElem0;

== matlab function arducopter/Lowpass2p/Lowpass Roll/Lowpass2p ==
  data: u input; y output; sampleFreq input; cutoffFreq input; delElem1 data_store_memory; delElem2 data_store_memory
function y = lowpass2p(u, sampleFreq, cutoffFreq)
% Lowpass filter of order two
% Source: LowPassFilter2p.cpp
global delElem1
global delElem2

% Calculate parameters: LowPassFilter2p.cpp, compute_params()
fr = single(sampleFreq/cutoffFreq);
ohm = single(tan(pi/fr));
c = single(1+2*cos(pi/4)*ohm + ohm*ohm);

b0 = ohm*ohm/c;
b1 = 2*b0;
b2 = b0;
a1 = 2*(ohm*ohm-1)/c;
a2 = single((1-2*cos(pi/4)*ohm+ohm*ohm)/c);

% Calculation of filtered sample: LowPassFilter2p.cpp, apply()
delElem0 = u - delElem1 * a1 - delElem2 * a2;
y = delElem0 * b0 + delElem1 * b1 + delElem2 * b2;

delElem2 = delElem1;
delElem1 = delElem0;
